simulink model "Robot_V11_DH_Torque"  (R2025b)
settings: Solver=ode1  StartTime=0.0  StopTime=2*T_ida+2*T_espera  FixedStep=0.001  RelTol=1e-3
InitFcn:
  | addpath(fileparts(which(bdroot)));
model workspace (MAT data in the model file):
  T_espera = 0.5
  T_ida = 2
undefined symbols (not defined in the file): X, Y, Z
libraries: sm_lib x28, nesl_utility x27, simulink x6
settings Model: Creator=nnavn  LastModifiedBy=nnavn

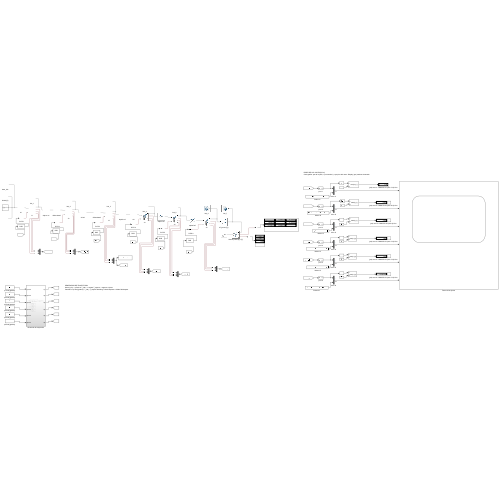
[thumbnail: Simulink's stored preview of the top-level diagram]
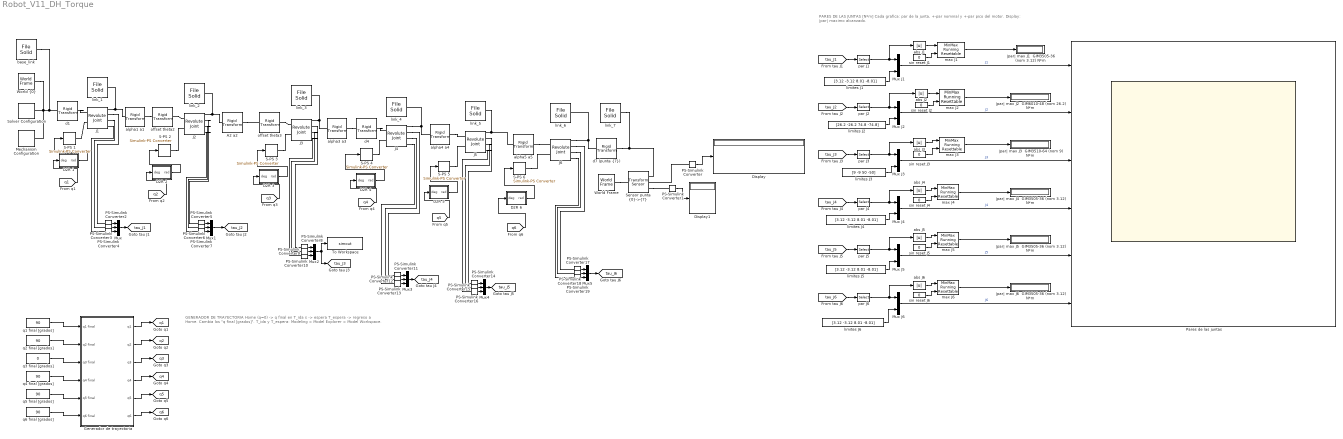
== system Robot_V11_DH_Torque ==
  note: GENERADOR DE TRAYECTORIA
      | Home (q=0) -> q final en T_ida s -> espera T_espera -> regreso a Home.
      | Cambia los "q final [grados]". T_ida y T_espera: Modeling > Model Explorer > Model Workspace.
  note: PARES DE LAS JUNTAS [N*m]
      | Cada grafica: par de la junta, +-par nominal y +-par pico del motor. Display: |par| maximo alcanzado.
  A2 a2 : sm_lib/Frames and Transforms/Rigid Transform  RotationMethod=None  FollAlignAxisA=+X  BaseAlignAxisA=+Y  FollAlignAxisB=+Y  BaseAlignAxisB=+Z  RotationStandardAxis=+Z  RotationAngle=0  RotationAngleUnits=deg  RotationArbitraryAxis=[0 0 1]  RotationSequenceAxes=FollowerAxes  RotationSequence=XYX  RotationSequenceAngles=[0 0 0]  RotationSequenceAnglesUnits=deg  RotationMatrix=[1 0 0;0 1 0;0 0 1]  Quaternion=[1 0 0 0]  TranslationMethod=StandardAxis  TranslationCartesianOffset=[0 0 0]  TranslationCartesianOffsetUnits=m  TranslationStandardAxis=+X  TranslationStandardOffset=0.16  TranslationStandardOffsetUnits=m  TranslationROffset=0  TranslationROffsetUnits=m  TranslationThetaOffset=0  TranslationThetaOffsetUnits=deg  TranslationZOffset=0  TranslationZOffsetUnits=m
  D2R 1 : Subsystem
      mask Display: disp('D2R')
  D2R 2 : Subsystem
      mask Display: disp('D2R')
  D2R 3 : Subsystem
      mask Display: disp('D2R')
  D2R 4 : Subsystem
      mask Display: disp('D2R')
  D2R 5 : Subsystem
      mask Display: disp('D2R')
  D2R 6 : Subsystem
      mask Display: disp('D2R')
  Display : Display
  Display1 : Display
  Generador de trayectoria : Subsystem
  J{1..6} (6 alike) : sm_lib/Joints/Revolute Joint  JointMode=Normal  CompositeWrenchDir=FollowerOnBase  CompositeWrenchFrame=BaseFrame  SenseConstraintForce=off  SenseConstraintTorque=off  SenseTotalForce=off  SenseTotalTorque=off  PositionTargetSpecify=off  PositionTargetPriority=High  PositionTargetValue=0  PositionTargetValueUnits=deg  VelocityTargetSpecify=off  VelocityTargetPriority=High  VelocityTargetValue=0  VelocityTargetValueUnits=deg/s  EquilibriumPosition=0  EquilibriumPositionUnits=deg  SpringStiffness=0  SpringStiffnessUnits=N*m/deg  DampingCoefficient=0  DampingCoefficientUnits=N*m/(deg/s)  LowerLimitSpecify=off  LowerLimitBound=-90  LowerLimitBoundUnits=deg  LowerLimitStiffness=1e4  LowerLimitStiffnessUnits=N*m/deg  LowerLimitDamping=10  LowerLimitDampingUnits=N*m/(deg/s)  LowerLimitTransitionRegionWidth=0.1  LowerLimitTransitionRegionWidthUnits=deg  UpperLimitSpecify=off  UpperLimitBound=90  UpperLimitBoundUnits=deg  UpperLimitStiffness=1e4  UpperLimitStiffnessUnits=N*m/deg  UpperLimitDamping=10  UpperLimitDampingUnits=N*m/(deg/s)  UpperLimitTransitionRegionWidth=0.1  UpperLimitTransitionRegionWidthUnits=deg  TorqueActuationMode=ComputedTorque  MotionActuationMode=InputMotion  SensePosition=off  SenseVelocity=off  SenseAcceleration=off  SenseTorqueForce=on  SenseLowerLimitTorqueForce=on  SenseUpperLimitTorqueForce=on
  Mechanism Configuration : sm_lib/Utilities/Mechanism Configuration  UniformGravity=Constant  GravityVector=[0 0 -9.81]  GravityVectorUnits=m/s^2  LinearizationDelta=0.001  JointModeTransitionNonlinearIterations=2
  Mux{,1..5} (6 alike) : Mux  Inputs=3
  Mux J{1..6} (6 alike) : Mux  Inputs=2
  PS-Simulink Converter{,1,3..4,6..7,9..10,12..13,15..16,18..19} (14 alike) : nesl_utility/PS-Simulink Converter  PhysicalDomain=network_engine_domain  SubClassName=ps_output  LeftPortType=input  RightPortType=output  PseudoPeriodic=off  Frequencies=[]  VectorFormat=inherit  Unit=inherit  AffineConversion=off
  PS-Simulink Converter{2,5,8,11,14,17} (6 alike) : nesl_utility/PS-Simulink Converter  PhysicalDomain=network_engine_domain  SubClassName=ps_output  LeftPortType=input  RightPortType=output  PseudoPeriodic=off  Frequencies=[]  VectorFormat=inherit  Unit=N*m  AffineConversion=off
  Pares de las juntas : Scope  NumInputPorts=6
      settings: ActiveDisplayString=6  Title="J6  GIM3505-36   nominal 3.12 / pico 8.01 N*m"  ActiveDisplayYMinimum=-9.2115  ActiveDisplayYMaximum=9.2115  YLabel=par [N*m]
  S-PS {1..6} (6 alike) : nesl_utility/Simulink-PS Converter  PhysicalDomain=network_engine_domain  SubClassName=ps_input  LeftPortType=input  RightPortType=output  PseudoPeriodic=off  Frequencies=[]  NoiseDistribution=none  NoiseParameters=[]  Unit=rad  AffineConversion=off  FilteringAndDerivatives=filter  SimscapeFilterOrder=2  InputFilterTimeConstant=0.01  UdotUserProvided=0
  "Sensor punta {0}->{7}" : sm_lib/Frames and Transforms/Transform Sensor  MeasurementFrame=World  RotationSequence=XYX  SenseAngle=off  SenseAxis=off  SenseQ=off  SenseR=on  SenseRotationSequence=off  SenseOmegaX=off  SenseOmegaY=off  SenseOmegaZ=off  SenseOmega=off  SenseQDot=off  SenseRDot=off  SenseRotationSequenceDot=off  SenseAlphaX=off  SenseAlphaY=off  SenseAlphaZ=off  SenseAlpha=off  SenseQDDot=off  SenseRDDot=off  SenseX=off  SenseY=off  SenseZ=off  SenseXYZ=on  SenseRad=off  SenseAzim=off  SenseDist=off  SenseInc=off  SenseXDot=off  SenseYDot=off  SenseZDot=off  SenseXYZDot=off  SenseRadDot=off  SenseAzimDot=off  SenseDistDot=off  SenseIncDot=off  SenseXDDot=off  SenseYDDot=off  SenseZDDot=off  SenseXYZDDot=off  SenseRadDDot=off  SenseAzimDDot=off  SenseDistDDot=off  SenseIncDDot=off
  Solver Configuration : nesl_utility/Solver Configuration  PhysicalDomain=network_engine_domain  SubClassName=solver  LeftPortType=input  RightPortType=generic  Tones=[]  Harmonics=[]  SimulateNoise=off  Profile=off  UseLocalSampling=off  EnableSwitchedLinearOptims=on  FrequencyDomain=off  UseCCode=off  RelTol=0.001  AbsTol=0.001  MinStep=1e-09  ToWorkspace=off  RevertToSquareIcSolve=off  NumHomotopyIterations=100  PhasorMode=off  PhasorModeNumHarmonics=1  ConsistencySolver=NEWTON_XTOL_AFTER_FTOL  IndexReductionMethod=DerivativeReplacement  DoDC=off  ResidualTolerance=1e-09  ConsistencyTolSource=GLOBAL  ConsistencyAbsTol=0.001  ConsistencyRelTol=0.001  ConsistencyTolFactor=0.001  UseLocalSolver=off  LocalSolverChoice=NE_BACKWARD_EULER_ADVANCER  ResolveIndetEquations=on  FunctionEvalNumThread=1  LocalSolverSampleTime=0.001  DoFixedCost=off  MaxNonlinIter=3  MaxModeIter=2  ComputeImpulses=off  ImpulseIterations=2  LinearAlgebra=auto  LinearAlgebraNumThread=0  EquationFormulation=NE_TIME_EF  DelaysMemoryBudget=1024  AutomaticFiltering=on  FilteringTimeConstant=0.001  PartitionStorageMethod=AS_NEEDED  PartitionMemoryBudget=1024  PartitionMethod=ROBUST  MultibodyUseLocalSolver=off  MultibodyLocalSolverChoice=ODE1  MultibodyLocalSolverSampleTime=0.001
  To Workspace : ToWorkspace  VariableName=simout  SampleTime=-1
  World Frame : sm_lib/Frames and Transforms/World Frame
  "World {0}" : sm_lib/Frames and Transforms/World Frame
  abs J{1..6} (6 alike) : Abs  SaturateOnIntegerOverflow=off
  alpha1 a1 : sm_lib/Frames and Transforms/Rigid Transform  RotationMethod=StandardAxis  FollAlignAxisA=+X  BaseAlignAxisA=+Y  FollAlignAxisB=+Y  BaseAlignAxisB=+Z  RotationStandardAxis=+X  RotationAngle=pi/2  RotationAngleUnits=rad  RotationArbitraryAxis=[0 0 1]  RotationSequenceAxes=FollowerAxes  RotationSequence=XYX  RotationSequenceAngles=[0 0 0]  RotationSequenceAnglesUnits=deg  RotationMatrix=[1 0 0;0 1 0;0 0 1]  Quaternion=[1 0 0 0]  TranslationMethod=None  TranslationCartesianOffset=[0 0 0]  TranslationCartesianOffsetUnits=m  TranslationStandardAxis=+Z  TranslationStandardOffset=0  TranslationStandardOffsetUnits=m  TranslationROffset=0  TranslationROffsetUnits=m  TranslationThetaOffset=0  TranslationThetaOffsetUnits=deg  TranslationZOffset=0  TranslationZOffsetUnits=m
  alpha3 a3 : sm_lib/Frames and Transforms/Rigid Transform  RotationMethod=StandardAxis  FollAlignAxisA=+X  BaseAlignAxisA=+Y  FollAlignAxisB=+Y  BaseAlignAxisB=+Z  RotationStandardAxis=-X  RotationAngle=pi/2  RotationAngleUnits=rad  RotationArbitraryAxis=[0 0 1]  RotationSequenceAxes=FollowerAxes  RotationSequence=XYX  RotationSequenceAngles=[0 0 0]  RotationSequenceAnglesUnits=deg  RotationMatrix=[1 0 0;0 1 0;0 0 1]  Quaternion=[1 0 0 0]  TranslationMethod=None  TranslationCartesianOffset=[0 0 0]  TranslationCartesianOffsetUnits=m  TranslationStandardAxis=+Z  TranslationStandardOffset=0  TranslationStandardOffsetUnits=m  TranslationROffset=0  TranslationROffsetUnits=m  TranslationThetaOffset=0  TranslationThetaOffsetUnits=deg  TranslationZOffset=0  TranslationZOffsetUnits=m
  alpha4 a4 : sm_lib/Frames and Transforms/Rigid Transform  RotationMethod=StandardAxis  FollAlignAxisA=+X  BaseAlignAxisA=+Y  FollAlignAxisB=+Y  BaseAlignAxisB=+Z  RotationStandardAxis=+X  RotationAngle=pi/2  RotationAngleUnits=rad  RotationArbitraryAxis=[0 0 1]  RotationSequenceAxes=FollowerAxes  RotationSequence=XYX  RotationSequenceAngles=[0 0 0]  RotationSequenceAnglesUnits=deg  RotationMatrix=[1 0 0;0 1 0;0 0 1]  Quaternion=[1 0 0 0]  TranslationMethod=None  TranslationCartesianOffset=[0 0 0]  TranslationCartesianOffsetUnits=m  TranslationStandardAxis=+Z  TranslationStandardOffset=0  TranslationStandardOffsetUnits=m  TranslationROffset=0  TranslationROffsetUnits=m  TranslationThetaOffset=0  TranslationThetaOffsetUnits=deg  TranslationZOffset=0  TranslationZOffsetUnits=m
  alpha5 a5 : sm_lib/Frames and Transforms/Rigid Transform  RotationMethod=StandardAxis  FollAlignAxisA=+X  BaseAlignAxisA=+Y  FollAlignAxisB=+Y  BaseAlignAxisB=+Z  RotationStandardAxis=-X  RotationAngle=pi/2  RotationAngleUnits=rad  RotationArbitraryAxis=[0 0 1]  RotationSequenceAxes=FollowerAxes  RotationSequence=XYX  RotationSequenceAngles=[0 0 0]  RotationSequenceAnglesUnits=deg  RotationMatrix=[1 0 0;0 1 0;0 0 1]  Quaternion=[1 0 0 0]  TranslationMethod=None  TranslationCartesianOffset=[0 0 0]  TranslationCartesianOffsetUnits=m  TranslationStandardAxis=+Z  TranslationStandardOffset=0  TranslationStandardOffsetUnits=m  TranslationROffset=0  TranslationROffsetUnits=m  TranslationThetaOffset=0  TranslationThetaOffsetUnits=deg  TranslationZOffset=0  TranslationZOffsetUnits=m
  base_link : sm_lib/Body Elements/File Solid  ExtGeomFileName=V11_base_link.step  UnitType=FromFile  ExtGeomFileUnits=m  StepReaderType=HEX  ExportConvexHullGeometry=off  InertiaType=Custom  BasedOnType=Mass  Density=1000  DensityUnits=kg/m^3  Mass=3.22978608  MassUnits=kg  CenterOfMass=[-0.00441761 0.00021358 0.04987356]  CenterOfMassUnits=m  MomentsOfInertia=[0.01456918 0.01547730 0.02259753]  MomentsOfInertiaUnits=kg*m^2  ProductsOfInertia=[0 0 0]  ProductsOfInertiaUnits=kg*m^2  GraphicType=FromGeometry  MarkerShape=Sphere  MarkerSize=10  GraphicVisPropType=SimpleVisualProperties  GraphicDiffuseColor=[0.5 0.5 0.5]  GraphicOpacity=1  GraphicSpecularColor=[0.5 0.5 0.5 1.0]  GraphicAmbientColor=[0.15 0.15 0.15 1.0]  GraphicEmissiveColor=[0.0 0.0 0.0 1.0]  GraphicShininess=75  DoExposeReferenceFrame=on  SerializedFrames=<Frames/>
  d1 : sm_lib/Frames and Transforms/Rigid Transform  RotationMethod=None  FollAlignAxisA=+X  BaseAlignAxisA=+Y  FollAlignAxisB=+Y  BaseAlignAxisB=+Z  RotationStandardAxis=+Z  RotationAngle=0  RotationAngleUnits=deg  RotationArbitraryAxis=[0 0 1]  RotationSequenceAxes=FollowerAxes  RotationSequence=XYX  RotationSequenceAngles=[0 0 0]  RotationSequenceAnglesUnits=deg  RotationMatrix=[1 0 0;0 1 0;0 0 1]  Quaternion=[1 0 0 0]  TranslationMethod=StandardAxis  TranslationCartesianOffset=[0 0 0]  TranslationCartesianOffsetUnits=m  TranslationStandardAxis=+Z  TranslationStandardOffset=0.224  TranslationStandardOffsetUnits=m  TranslationROffset=0  TranslationROffsetUnits=m  TranslationThetaOffset=0  TranslationThetaOffsetUnits=deg  TranslationZOffset=0  TranslationZOffsetUnits=m
  d4 : sm_lib/Frames and Transforms/Rigid Transform  RotationMethod=None  FollAlignAxisA=+X  BaseAlignAxisA=+Y  FollAlignAxisB=+Y  BaseAlignAxisB=+Z  RotationStandardAxis=+Z  RotationAngle=0  RotationAngleUnits=deg  RotationArbitraryAxis=[0 0 1]  RotationSequenceAxes=FollowerAxes  RotationSequence=XYX  RotationSequenceAngles=[0 0 0]  RotationSequenceAnglesUnits=deg  RotationMatrix=[1 0 0;0 1 0;0 0 1]  Quaternion=[1 0 0 0]  TranslationMethod=StandardAxis  TranslationCartesianOffset=[0 0 0]  TranslationCartesianOffsetUnits=m  TranslationStandardAxis=+Z  TranslationStandardOffset=0.16  TranslationStandardOffsetUnits=m  TranslationROffset=0  TranslationROffsetUnits=m  TranslationThetaOffset=0  TranslationThetaOffsetUnits=deg  TranslationZOffset=0  TranslationZOffsetUnits=m
  "d7 (punta {7})" : sm_lib/Frames and Transforms/Rigid Transform  RotationMethod=None  FollAlignAxisA=+X  BaseAlignAxisA=+Y  FollAlignAxisB=+Y  BaseAlignAxisB=+Z  RotationStandardAxis=+Z  RotationAngle=0  RotationAngleUnits=deg  RotationArbitraryAxis=[0 0 1]  RotationSequenceAxes=FollowerAxes  RotationSequence=XYX  RotationSequenceAngles=[0 0 0]  RotationSequenceAnglesUnits=deg  RotationMatrix=[1 0 0;0 1 0;0 0 1]  Quaternion=[1 0 0 0]  TranslationMethod=StandardAxis  TranslationCartesianOffset=[0 0 0]  TranslationCartesianOffsetUnits=m  TranslationStandardAxis=+Z  TranslationStandardOffset=0.085  TranslationStandardOffsetUnits=m  TranslationROffset=0  TranslationROffsetUnits=m  TranslationThetaOffset=0  TranslationThetaOffsetUnits=deg  TranslationZOffset=0  TranslationZOffsetUnits=m
  limites J{1,4..6} (4 alike) : Constant  Value=[3.12 -3.12 8.01 -8.01]
  limites J2 : Constant  Value=[26.2 -26.2 74.8 -74.8]
  limites J3 : Constant  Value=[9 -9 50 -50]
  link_1 : sm_lib/Body Elements/File Solid  ExtGeomFileName=V11_link_1.step  UnitType=FromFile  ExtGeomFileUnits=m  StepReaderType=HEX  ExportConvexHullGeometry=off  InertiaType=Custom  BasedOnType=Mass  Density=1000  DensityUnits=kg/m^3  Mass=1.42277105  MassUnits=kg  CenterOfMass=|  CenterOfMassUnits=m  MomentsOfInertia=[0.00355071 0.00349208 0.00176143]  MomentsOfInertiaUnits=kg*m^2  ProductsOfInertia=[0 0 0]  ProductsOfInertiaUnits=kg*m^2  GraphicType=FromGeometry  MarkerShape=Sphere  MarkerSize=10  GraphicVisPropType=SimpleVisualProperties  GraphicDiffuseColor=[0.5 0.5 0.5]  GraphicOpacity=1  GraphicSpecularColor=[0.5 0.5 0.5 1.0]  GraphicAmbientColor=[0.15 0.15 0.15 1.0]  GraphicEmissiveColor=[0.0 0.0 0.0 1.0]  GraphicShininess=75  DoExposeReferenceFrame=on  SerializedFrames=<Frames/>
      | [0.00002116 -0.00249327 -0.02470983
      | ]
  link_2 : sm_lib/Body Elements/File Solid  ExtGeomFileName=V11_link_2.step  UnitType=FromFile  ExtGeomFileUnits=m  StepReaderType=HEX  ExportConvexHullGeometry=off  InertiaType=Custom  BasedOnType=Mass  Density=1000  DensityUnits=kg/m^3  Mass=1.25185199  MassUnits=kg  CenterOfMass=[0.00211573 0.00696012 0.00548348]  CenterOfMassUnits=m  MomentsOfInertia=[0.00211573 0.00696012 0.00548348]  MomentsOfInertiaUnits=kg*m^2  ProductsOfInertia=[0 0 0]  ProductsOfInertiaUnits=kg*m^2  GraphicType=FromGeometry  MarkerShape=Sphere  MarkerSize=10  GraphicVisPropType=SimpleVisualProperties  GraphicDiffuseColor=[0.5 0.5 0.5]  GraphicOpacity=1  GraphicSpecularColor=[0.5 0.5 0.5 1.0]  GraphicAmbientColor=[0.15 0.15 0.15 1.0]  GraphicEmissiveColor=[0.0 0.0 0.0 1.0]  GraphicShininess=75  DoExposeReferenceFrame=on  SerializedFrames=<Frames/>
  link_3 : sm_lib/Body Elements/File Solid  ExtGeomFileName=V11_link_3.step  UnitType=FromFile  ExtGeomFileUnits=m  StepReaderType=HEX  ExportConvexHullGeometry=off  InertiaType=Custom  BasedOnType=Mass  Density=1000  DensityUnits=kg/m^3  Mass=0.58966599  MassUnits=kg  CenterOfMass=|  CenterOfMassUnits=m  MomentsOfInertia=|  MomentsOfInertiaUnits=kg*m^2  ProductsOfInertia=[0 0 0]  ProductsOfInertiaUnits=kg*m^2  GraphicType=FromGeometry  MarkerShape=Sphere  MarkerSize=10  GraphicVisPropType=SimpleVisualProperties  GraphicDiffuseColor=[0.5 0.5 0.5]  GraphicOpacity=1  GraphicSpecularColor=[0.5 0.5 0.5 1.0]  GraphicAmbientColor=[0.15 0.15 0.15 1.0]  GraphicEmissiveColor=[0.0 0.0 0.0 1.0]  GraphicShininess=75  DoExposeReferenceFrame=on  SerializedFrames=<Frames/>
      CenterOfMass=|
      | [ -0.00009416
      |  0.04213010
      |  -0.00460755]
      MomentsOfInertia=|
      | [0.00170461 0.00133106 0.00063002
      | ]
  link_4 : sm_lib/Body Elements/File Solid  ExtGeomFileName=V11_link_4.step  UnitType=FromFile  ExtGeomFileUnits=m  StepReaderType=HEX  ExportConvexHullGeometry=off  InertiaType=Custom  BasedOnType=Mass  Density=1000  DensityUnits=kg/m^3  Mass=0.47958111  MassUnits=kg  CenterOfMass=|  CenterOfMassUnits=m  MomentsOfInertia="[0.00072785  0.00066618 0.00040986]"  MomentsOfInertiaUnits=kg*m^2  ProductsOfInertia=[0 0 0]  ProductsOfInertiaUnits=kg*m^2  GraphicType=FromGeometry  MarkerShape=Sphere  MarkerSize=10  GraphicVisPropType=SimpleVisualProperties  GraphicDiffuseColor=[0.5 0.5 0.5]  GraphicOpacity=1  GraphicSpecularColor=[0.5 0.5 0.5 1.0]  GraphicAmbientColor=[0.15 0.15 0.15 1.0]  GraphicEmissiveColor=[0.0 0.0 0.0 1.0]  GraphicShininess=75  DoExposeReferenceFrame=on  SerializedFrames=<Frames/>
      | [-0.00008520
      | -0.00067765
      | -0.02985032]
  link_5 : sm_lib/Body Elements/File Solid  ExtGeomFileName=V11_link_5.step  UnitType=FromFile  ExtGeomFileUnits=m  StepReaderType=HEX  ExportConvexHullGeometry=off  InertiaType=Custom  BasedOnType=Mass  Density=1000  DensityUnits=kg/m^3  Mass=0.44332189  MassUnits=kg  CenterOfMass=|  CenterOfMassUnits=m  MomentsOfInertia=[0.00057612 0.00037214 0.00034469]  MomentsOfInertiaUnits=kg*m^2  ProductsOfInertia=[0 0 0]  ProductsOfInertiaUnits=kg*m^2  GraphicType=FromGeometry  MarkerShape=Sphere  MarkerSize=10  GraphicVisPropType=SimpleVisualProperties  GraphicDiffuseColor=[0.5 0.5 0.5]  GraphicOpacity=1  GraphicSpecularColor=[0.5 0.5 0.5 1.0]  GraphicAmbientColor=[0.15 0.15 0.15 1.0]  GraphicEmissiveColor=[0.0 0.0 0.0 1.0]  GraphicShininess=75  DoExposeReferenceFrame=on  SerializedFrames=<Frames/>
      | [ -0.00010871
      | 0.03642818
      | -0.00232872]
  link_6 : sm_lib/Body Elements/File Solid  ExtGeomFileName=V11_link_6.step  UnitType=FromFile  ExtGeomFileUnits=m  StepReaderType=HEX  ExportConvexHullGeometry=off  InertiaType=Custom  BasedOnType=Mass  Density=1000  DensityUnits=kg/m^3  Mass=0.05458529  MassUnits=kg  CenterOfMass=|  CenterOfMassUnits=m  MomentsOfInertia=[0.00001352 0.00001352 0.00002663]  MomentsOfInertiaUnits=kg*m^2  ProductsOfInertia=[0 0 0]  ProductsOfInertiaUnits=kg*m^2  GraphicType=FromGeometry  MarkerShape=Sphere  MarkerSize=10  GraphicVisPropType=SimpleVisualProperties  GraphicDiffuseColor=[0.5 0.5 0.5]  GraphicOpacity=1  GraphicSpecularColor=[0.5 0.5 0.5 1.0]  GraphicAmbientColor=[0.15 0.15 0.15 1.0]  GraphicEmissiveColor=[0.0 0.0 0.0 1.0]  GraphicShininess=75  DoExposeReferenceFrame=on  SerializedFrames=<Frames/>
      | [0.00000000
      | 0.00000000
      | 0.08009328]
  link_7 : sm_lib/Body Elements/File Solid  ExtGeomFileName=V11_link_6.step  UnitType=FromFile  ExtGeomFileUnits=m  StepReaderType=HEX  ExportConvexHullGeometry=off  InertiaType=Custom  BasedOnType=Mass  Density=1000  DensityUnits=kg/m^3  Mass=1  MassUnits=kg  CenterOfMass=|  CenterOfMassUnits=m  MomentsOfInertia=[0.00001352 0.00001352 0.00002663]  MomentsOfInertiaUnits=kg*m^2  ProductsOfInertia=[0 0 0]  ProductsOfInertiaUnits=kg*m^2  GraphicType=FromGeometry  MarkerShape=Sphere  MarkerSize=10  GraphicVisPropType=SimpleVisualProperties  GraphicDiffuseColor=[0.5 0.5 0.5]  GraphicOpacity=1  GraphicSpecularColor=[0.5 0.5 0.5 1.0]  GraphicAmbientColor=[0.15 0.15 0.15 1.0]  GraphicEmissiveColor=[0.0 0.0 0.0 1.0]  GraphicShininess=75  DoExposeReferenceFrame=on  SerializedFrames=<Frames/>
      | [0.00000000
      | 0.00000000
      | 0.08009328]
  max J{1..6} (6 alike) : simulink/Math Operations/MinMax Running Resettable  Function=max  vinit=0.0
  offset theta2 : sm_lib/Frames and Transforms/Rigid Transform  RotationMethod=StandardAxis  FollAlignAxisA=+X  BaseAlignAxisA=+Y  FollAlignAxisB=+Y  BaseAlignAxisB=+Z  RotationStandardAxis=+Z  RotationAngle=pi/2  RotationAngleUnits=rad  RotationArbitraryAxis=[0 0 1]  RotationSequenceAxes=FollowerAxes  RotationSequence=XYX  RotationSequenceAngles=[0 0 0]  RotationSequenceAnglesUnits=deg  RotationMatrix=[1 0 0;0 1 0;0 0 1]  Quaternion=[1 0 0 0]  TranslationMethod=None  TranslationCartesianOffset=[0 0 0]  TranslationCartesianOffsetUnits=m  TranslationStandardAxis=+Z  TranslationStandardOffset=0  TranslationStandardOffsetUnits=m  TranslationROffset=0  TranslationROffsetUnits=m  TranslationThetaOffset=0  TranslationThetaOffsetUnits=deg  TranslationZOffset=0  TranslationZOffsetUnits=m
  offset theta3 : sm_lib/Frames and Transforms/Rigid Transform  RotationMethod=StandardAxis  FollAlignAxisA=+X  BaseAlignAxisA=+Y  FollAlignAxisB=+Y  BaseAlignAxisB=+Z  RotationStandardAxis=-Z  RotationAngle=pi/2  RotationAngleUnits=rad  RotationArbitraryAxis=[0 0 1]  RotationSequenceAxes=FollowerAxes  RotationSequence=XYX  RotationSequenceAngles=[0 0 0]  RotationSequenceAnglesUnits=deg  RotationMatrix=[1 0 0;0 1 0;0 0 1]  Quaternion=[1 0 0 0]  TranslationMethod=None  TranslationCartesianOffset=[0 0 0]  TranslationCartesianOffsetUnits=m  TranslationStandardAxis=+Z  TranslationStandardOffset=0  TranslationStandardOffsetUnits=m  TranslationROffset=0  TranslationROffsetUnits=m  TranslationThetaOffset=0  TranslationThetaOffsetUnits=deg  TranslationZOffset=0  TranslationZOffsetUnits=m
  par J{1..6} (6 alike) : Selector  InputPortWidth=3  IndexOptions=Index vector (dialog)  Indices=1  OutputSizes=1
  q1 final [grados] : Constant  Value=90
  q2 final [grados] : Constant  Value=90
  q3 final [grados] : Constant  Value=0
  q4 final [grados] : Constant  Value=90
  q5 final [grados] : Constant  Value=90
  q6 final [grados] : Constant  Value=90
  sin reset J{1..6} (6 alike) : Constant  Value=0
  |par| max J1  GIM3505-36 (nom 3.12) N*m : Display
  |par| max J2  GIM6010-48 (nom 26.2) N*m : Display
  |par| max J3  GIM3510-64 (nom 9) N*m : Display
  |par| max J4  GIM3505-36 (nom 3.12) N*m : Display
  |par| max J5  GIM3505-36 (nom 3.12) N*m : Display
  |par| max J6  GIM3505-36 (nom 3.12) N*m : Display
  tag scope: q1=global, q2=global, q3=global, q4=global, q5=global, q6=global, tau_J1=global, tau_J2=global, tau_J3=global, tau_J4=global, tau_J5=global, tau_J6=global
  wires:
  D2R 1/1(rad) -> S-PS 1/1
  D2R 2/1(rad) -> S-PS 2/1
  D2R 3/1(rad) -> S-PS 3/1
  D2R 4/1(rad) -> S-PS 4/1
  D2R 5/1(rad) -> S-PS 5/1
  D2R 6/1(rad) -> S-PS 6/1
  PS-Simulink Converter1/1 -> Display1/1
  PS-Simulink Converter/1 -> Display/1
  PS-Simulink Converter4/1 -> Mux/3
  PS-Simulink Converter3/1 -> Mux/2
  PS-Simulink Converter2/1 -> Mux/1
  PS-Simulink Converter7/1 -> Mux1/3
  PS-Simulink Converter6/1 -> Mux1/2
  PS-Simulink Converter5/1 -> Mux1/1
  Mux2/1 -> To Workspace/1, [tau_J3]
  PS-Simulink Converter9/1 -> Mux2/2
  PS-Simulink Converter10/1 -> Mux2/3
  PS-Simulink Converter8/1 -> Mux2/1
  PS-Simulink Converter12/1 -> Mux3/2
  PS-Simulink Converter13/1 -> Mux3/3
  PS-Simulink Converter11/1 -> Mux3/1
  PS-Simulink Converter15/1 -> Mux4/2
  PS-Simulink Converter16/1 -> Mux4/3
  PS-Simulink Converter14/1 -> Mux4/1
  PS-Simulink Converter18/1 -> Mux5/2
  PS-Simulink Converter19/1 -> Mux5/3
  PS-Simulink Converter17/1 -> Mux5/1
  [q1] -> D2R 1/1(deg)
  [q2] -> D2R 2/1(deg)
  [q3] -> D2R 3/1(deg)
  [q4] -> D2R 4/1(deg)
  [q5] -> D2R 5/1(deg)
  [q6] -> D2R 6/1(deg)
  Mux/1 -> [tau_J1]
  Mux1/1 -> [tau_J2]
  Mux3/1 -> [tau_J4]
  Mux4/1 -> [tau_J5]
  Mux5/1 -> [tau_J6]
  q1 final [grados]/1 -> Generador de trayectoria/1(q1 final)
  Generador de trayectoria/1(q1) -> [q1]
  q2 final [grados]/1 -> Generador de trayectoria/2(q2 final)
  Generador de trayectoria/2(q2) -> [q2]
  q3 final [grados]/1 -> Generador de trayectoria/3(q3 final)
  Generador de trayectoria/3(q3) -> [q3]
  q4 final [grados]/1 -> Generador de trayectoria/4(q4 final)
  Generador de trayectoria/4(q4) -> [q4]
  q5 final [grados]/1 -> Generador de trayectoria/5(q5 final)
  Generador de trayectoria/5(q5) -> [q5]
  q6 final [grados]/1 -> Generador de trayectoria/6(q6 final)
  Generador de trayectoria/6(q6) -> [q6]
  [tau_J1] -> par J1/1
  par J1/1 -> Mux J1/1, abs J1/1
  limites J1/1 -> Mux J1/2
  abs J1/1 -> max J1/1
  sin reset J1/1 -> max J1/2
  max J1/1 -> |par| max J1  GIM3505-36 (nom 3.12) N*m/1
  Mux J1/1 -> Pares de las juntas/1  "J1"
  [tau_J2] -> par J2/1
  par J2/1 -> Mux J2/1, abs J2/1
  limites J2/1 -> Mux J2/2
  abs J2/1 -> max J2/1
  sin reset J2/1 -> max J2/2
  max J2/1 -> |par| max J2  GIM6010-48 (nom 26.2) N*m/1
  Mux J2/1 -> Pares de las juntas/2  "J2"
  [tau_J3] -> par J3/1
  par J3/1 -> Mux J3/1, abs J3/1
  limites J3/1 -> Mux J3/2
  abs J3/1 -> max J3/1
  sin reset J3/1 -> max J3/2
  max J3/1 -> |par| max J3  GIM3510-64 (nom 9) N*m/1
  Mux J3/1 -> Pares de las juntas/3  "J3"
  [tau_J4] -> par J4/1
  par J4/1 -> Mux J4/1, abs J4/1
  limites J4/1 -> Mux J4/2
  abs J4/1 -> max J4/1
  sin reset J4/1 -> max J4/2
  max J4/1 -> |par| max J4  GIM3505-36 (nom 3.12) N*m/1
  Mux J4/1 -> Pares de las juntas/4  "J4"
  [tau_J5] -> par J5/1
  par J5/1 -> Mux J5/1, abs J5/1
  limites J5/1 -> Mux J5/2
  abs J5/1 -> max J5/1
  sin reset J5/1 -> max J5/2
  max J5/1 -> |par| max J5  GIM3505-36 (nom 3.12) N*m/1
  Mux J5/1 -> Pares de las juntas/5  "J5"
  [tau_J6] -> par J6/1
  par J6/1 -> Mux J6/1, abs J6/1
  limites J6/1 -> Mux J6/2
  abs J6/1 -> max J6/1
  sin reset J6/1 -> max J6/2
  max J6/1 -> |par| max J6  GIM3505-36 (nom 3.12) N*m/1
  Mux J6/1 -> Pares de las juntas/6  "J6"
  connections:
  Solver Configuration/RConn1 -- "World {0}"/RConn1 -- Mechanism Configuration/RConn1 -- base_link/RConn1 -- d1/LConn1
  d1/RConn1 -- J1/LConn1
  J1/RConn1 -- alpha1 a1/LConn1 -- link_1/RConn1
  S-PS 1/RConn1 -- J1/LConn2
  alpha1 a1/RConn1 -- offset theta2/LConn1
  offset theta2/RConn1 -- J2/LConn1
  J2/RConn1 -- A2 a2/LConn1 -- link_2/RConn1
  S-PS 2/RConn1 -- J2/LConn2
  A2 a2/RConn1 -- offset theta3/LConn1
  offset theta3/RConn1 -- J3/LConn1
  J3/RConn1 -- alpha3 a3/LConn1 -- link_3/RConn1
  S-PS 3/RConn1 -- J3/LConn2
  alpha3 a3/RConn1 -- d4/LConn1
  d4/RConn1 -- J4/LConn1
  J4/RConn1 -- alpha4 a4/LConn1 -- link_4/RConn1
  S-PS 4/RConn1 -- J4/LConn2
  alpha4 a4/RConn1 -- J5/LConn1
  S-PS 5/RConn1 -- J5/LConn2
  alpha5 a5/RConn1 -- J6/LConn1
  J6/RConn1 -- "d7 (punta {7})"/LConn1 -- link_6/RConn1
  S-PS 6/RConn1 -- J6/LConn2
  "d7 (punta {7})"/RConn1 -- link_7/RConn1 -- "Sensor punta {0}->{7}"/RConn1
  link_5/RConn1 -- alpha5 a5/LConn1 -- J5/RConn1
  PS-Simulink Converter/LConn1 -- "Sensor punta {0}->{7}"/RConn2
  "Sensor punta {0}->{7}"/RConn3 -- PS-Simulink Converter1/LConn1
  World Frame/RConn1 -- "Sensor punta {0}->{7}"/LConn1
  J1/RConn2 -- PS-Simulink Converter2/LConn1
  J1/RConn3 -- PS-Simulink Converter3/LConn1
  J1/RConn4 -- PS-Simulink Converter4/LConn1
  J6/RConn2 -- PS-Simulink Converter17/LConn1
  J6/RConn3 -- PS-Simulink Converter18/LConn1
  J6/RConn4 -- PS-Simulink Converter19/LConn1
  J5/RConn2 -- PS-Simulink Converter14/LConn1
  J5/RConn3 -- PS-Simulink Converter15/LConn1
  J5/RConn4 -- PS-Simulink Converter16/LConn1
  J4/RConn2 -- PS-Simulink Converter11/LConn1
  J4/RConn3 -- PS-Simulink Converter12/LConn1
  J4/RConn4 -- PS-Simulink Converter13/LConn1
  J3/RConn2 -- PS-Simulink Converter8/LConn1
  J3/RConn3 -- PS-Simulink Converter9/LConn1
  J3/RConn4 -- PS-Simulink Converter10/LConn1
  J2/RConn2 -- PS-Simulink Converter5/LConn1
  J2/RConn3 -- PS-Simulink Converter6/LConn1
  J2/RConn4 -- PS-Simulink Converter7/LConn1

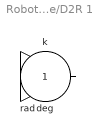
== system Robot_V11_DH_Torque/D2R 1 ==
  deg : Inport
  k : Gain  Gain=pi/180
  rad : Outport
  wires:
  deg/1 -> k/1
  k/1 -> rad/1

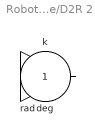
== system Robot_V11_DH_Torque/D2R 2 ==
  deg : Inport
  k : Gain  Gain=pi/180
  rad : Outport
  wires:
  deg/1 -> k/1
  k/1 -> rad/1

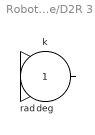
== system Robot_V11_DH_Torque/D2R 3 ==
  deg : Inport
  k : Gain  Gain=pi/180
  rad : Outport
  wires:
  deg/1 -> k/1
  k/1 -> rad/1

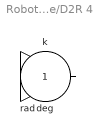
== system Robot_V11_DH_Torque/D2R 4 ==
  deg : Inport
  k : Gain  Gain=pi/180
  rad : Outport
  wires:
  deg/1 -> k/1
  k/1 -> rad/1

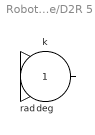
== system Robot_V11_DH_Torque/D2R 5 ==
  deg : Inport
  k : Gain  Gain=pi/180
  rad : Outport
  wires:
  deg/1 -> k/1
  k/1 -> rad/1

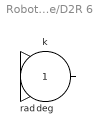
== system Robot_V11_DH_Torque/D2R 6 ==
  deg : Inport
  k : Gain  Gain=pi/180
  rad : Outport
  wires:
  deg/1 -> k/1
  k/1 -> rad/1

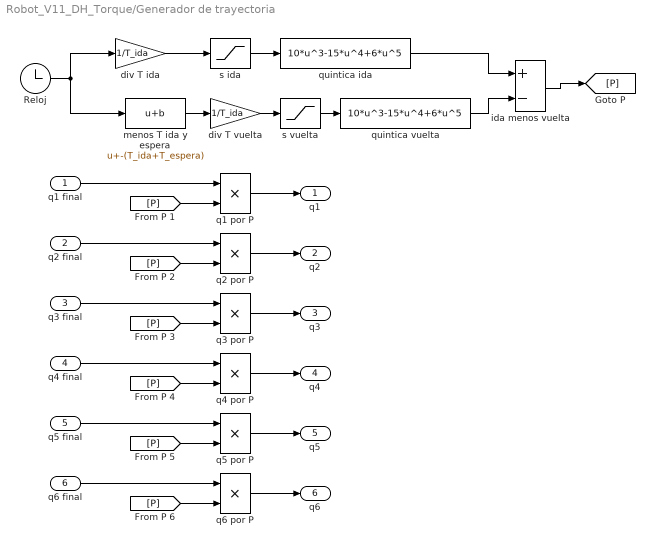
== system Robot_V11_DH_Torque/Generador de trayectoria ==
  q1 final : Inport
  q2 final : Inport  Port=2
  q3 final : Inport  Port=3
  q4 final : Inport  Port=4
  q5 final : Inport  Port=5
  q6 final : Inport  Port=6
  Reloj : Clock
  div T ida : Gain  Gain=1/T_ida
  div T vuelta : Gain  Gain=1/T_ida
  ida menos vuelta : Sum  Inputs=+-
  menos T ida y espera : Bias  Bias=-(T_ida+T_espera)  SaturateOnIntegerOverflow=off
  q1 por P : Product
  q2 por P : Product
  q3 por P : Product
  q4 por P : Product
  q5 por P : Product
  q6 por P : Product
  quintica ida : Fcn  Expr=10*u^3-15*u^4+6*u^5
  quintica vuelta : Fcn  Expr=10*u^3-15*u^4+6*u^5
  s ida : Saturate  UpperLimit=1  LowerLimit=0
  s vuelta : Saturate  UpperLimit=1  LowerLimit=0
  q1 : Outport
  q2 : Outport  Port=2
  q3 : Outport  Port=3
  q4 : Outport  Port=4
  q5 : Outport  Port=5
  q6 : Outport  Port=6
  wires:
  Reloj/1 -> div T ida/1, menos T ida y espera/1
  div T ida/1 -> s ida/1
  s ida/1 -> quintica ida/1
  menos T ida y espera/1 -> div T vuelta/1
  div T vuelta/1 -> s vuelta/1
  s vuelta/1 -> quintica vuelta/1
  quintica ida/1 -> ida menos vuelta/1
  quintica vuelta/1 -> ida menos vuelta/2
  ida menos vuelta/1 -> [P]
  q1 final/1 -> q1 por P/1
  [P] -> q1 por P/2
  q1 por P/1 -> q1/1
  q2 final/1 -> q2 por P/1
  [P] -> q2 por P/2
  q2 por P/1 -> q2/1
  q3 final/1 -> q3 por P/1
  [P] -> q3 por P/2
  q3 por P/1 -> q3/1
  q4 final/1 -> q4 por P/1
  [P] -> q4 por P/2
  q4 por P/1 -> q4/1
  q5 final/1 -> q5 por P/1
  [P] -> q5 por P/2
  q5 por P/1 -> q5/1
  q6 final/1 -> q6 por P/1
  [P] -> q6 por P/2
  q6 por P/1 -> q6/1
